simulink model "sm_car"  (R2025a)
settings: Solver=ode23t  StartTime=0.0  StopTime=400  MaxStep=0.4  RelTol=1e-3  AbsTol=1e-3  EnableMultiTasking=on
PreLoadFcn:
  | % Due to usability issue in Repeating Sequence block
  | warning('off','Simulink:Masking:Invalid');
  | 
  | % Eliminate unnecessary warnings in inactive variants
  | % Warnings generated only if you click through inactive variant
  | warning('off','MATLAB:nonExistentField');
  | warning('off','Simulink:Parameters:BlkParamUndefined');
PostLoadFcn:
  | set_param([bdroot '/Vehicle'],'popup_trailer','Off')
  | warning('off','sm:sli:setup:compile:LocalSolverNotSupported')
  | %sm_car_config_maneuver(bdroot,'WOT Braking');
  | sm_car_config_vehicle(bdroot,'false');
  | sm_car_config_logging(bdroot);
InitFcn:
  | sm_car_config_camera;
  | Vehicle = sm_car_vehcfg_checkConfig(Vehicle);
  | sm_car_check_tire_model(bdroot);
StartFcn:
  | tic;
StopFcn:
  | Elapsed_Sim_Time = toc;
  | % disp(['Elapsed Sim Time = ' num2str(Elapsed_Sim_Time)]);
undefined symbols (not defined in the file): Axle1D, AxleIn, Camera, Control, Driver, Free, Init, Maneuver, Pedal, RaceFix, RaceSpin, Scene, ShaftL1, ShaftL2, ShaftR1, ShaftR2, Soft, Stiff, Visual, X, xy_data_car_side, Y, Z
libraries: sm_lib x1546, nesl_utility x528, fl_lib x480, SimscapeFluids_lib x61, sdl_lib x49, simulink x29, ee_lib x7, simulink_extras x6, Linkage_Systems x4, Tire_1x2x x4, AntiRollBar_Systems x2, Linkage_Decoupled x2
(part 28 of 79)

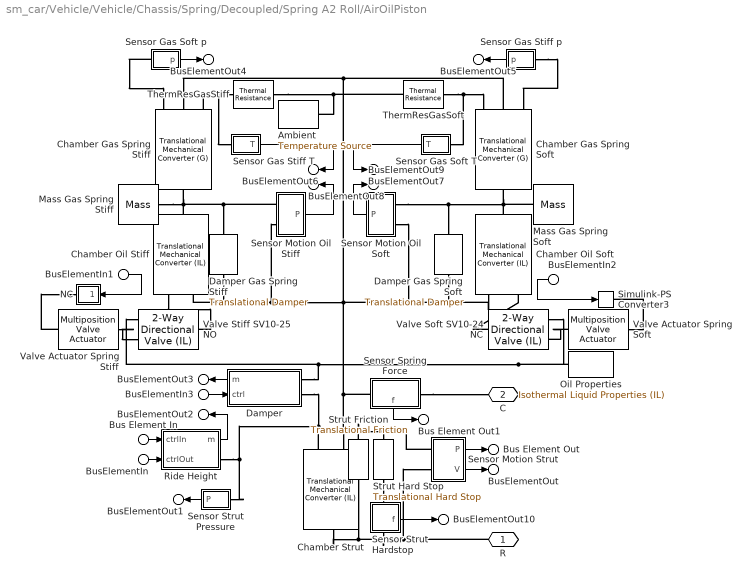
== system sm_car/Vehicle/Vehicle/Chassis/Spring/Decoupled/Spring A2 Roll/AirOilPiston ==
  BusElementIn1 : Inport  PortName=Ctrl  Element=GasSprStiff
  BusElementIn2 : Inport  PortName=Ctrl  Element=GasSprSoft
  BusElementIn3 : Inport  PortName=Ctrl  Element=Damper
  Bus Element In : Inport  PortName=Ctrl  Element=RideHeightIn
  BusElementIn : Inport  PortName=Ctrl  Element=RideHeightOut
  Ambient : fl_lib/Thermal/Thermal Sources/Temperature Source  temperature=t_ambient K
  Chamber Gas Spring Soft : fl_lib/Gas/Elements/Translational Mechanical Converter (G)  mech_orientation=foundation.enum.MechOrientationTranslational.Negative  displacement_spec=foundation.enum.DisplacementSpec.Calculate  length_init=gas_chamber_soft_x0 m  interface_area=gas_chamber_soft_area m^2  dead_volume=gas_chamber_soft_deadvol l  area_A=0.01 m^2  environment_spec=foundation.enum.pressure_spec.atmospheric  environment_pressure=0.101325 MPa  p_I_specify=on  p_I_priority=High  p_I=gas_chamber_soft_p0 MPa  p_I_nominal_specify=off  p_I_nominal_value=1  p_I_nominal_unit=MPa  T_I_specify=off  T_I_priority=High  T_I=293.15 K  T_I_nominal_specify=off  T_I_nominal_value=1  T_I_nominal_unit=K  rho_I_specify=off  rho_I_priority=None  rho_I=1.2 kg/m^3  rho_I_nominal_specify=off  rho_I_nominal_value=1  rho_I_nominal_unit=kg/m^3
      settings: InternalSimscapePortConfiguration="{\"Bottom\":[],\"Left\":[{\"id\":\"A\",\"label\":\"A\",\"type\":\"foundation.gas.gas\"},{\"id\":\"C\",\"label\":\"C\",\"type\":\"foundation.mechanical.translational.translational\"},{\"id\":\"H\",\"label\":\"H\",\"type\":\"foundation.thermal.thermal\"}],\"Right\":[{\"id\":\"R\",\"label\":\"R\",\"type\":\"foundation.mechanical.translational.translational\"}],\"Top\":[]}"
  Chamber Gas Spring Stiff : fl_lib/Gas/Elements/Translational Mechanical Converter (G)  mech_orientation=foundation.enum.MechOrientationTranslational.Negative  displacement_spec=foundation.enum.DisplacementSpec.Calculate  length_init=gas_chamber_stiff_x0 m  interface_area=gas_chamber_stiff_area m^2  dead_volume=gas_chamber_stiff_deadvol l  area_A=0.01 m^2  environment_spec=foundation.enum.pressure_spec.atmospheric  environment_pressure=0.101325 MPa  p_I_specify=on  p_I_priority=High  p_I=gas_chamber_stiff_p0 MPa  p_I_nominal_specify=off  p_I_nominal_value=1  p_I_nominal_unit=MPa  T_I_specify=off  T_I_priority=High  T_I=293.15 K  T_I_nominal_specify=off  T_I_nominal_value=1  T_I_nominal_unit=K  rho_I_specify=off  rho_I_priority=None  rho_I=1.2 kg/m^3  rho_I_nominal_specify=off  rho_I_nominal_value=1  rho_I_nominal_unit=kg/m^3
      settings: InternalSimscapePortConfiguration="{\"Bottom\":[],\"Left\":[{\"id\":\"A\",\"label\":\"A\",\"type\":\"foundation.gas.gas\"},{\"id\":\"C\",\"label\":\"C\",\"type\":\"foundation.mechanical.translational.translational\"},{\"id\":\"H\",\"label\":\"H\",\"type\":\"foundation.thermal.thermal\"}],\"Right\":[{\"id\":\"R\",\"label\":\"R\",\"type\":\"foundation.mechanical.translational.translational\"}],\"Top\":[]}"
  Chamber Oil Soft : fl_lib/Isothermal Liquid/Elements/Translational Mechanical Converter (IL)  mech_orientation=foundation.enum.MechOrientationTranslational.Positive  displacement_spec=foundation.enum.DisplacementSpec.Calculate  x0=oil_chamber_soft_x0 m  interface_area=oil_chamber_soft_area m^2  dead_volume=oil_chamber_soft_deadvol l  pressure_spec=foundation.enum.pressure_spec.atmospheric  environment_pressure=0.101325 MPa  dynamic_compressibility=simscape.enum.onoff.off  p0=Spring.Spring.OilSoft.pInit.Value MPa  p_nominal=0.101325 MPa
      settings: InternalSimscapePortConfiguration="{\"Bottom\":[],\"Left\":[{\"id\":\"A\",\"label\":\"A\",\"type\":\"foundation.isothermal_liquid.isothermal_liquid\"},{\"id\":\"C\",\"label\":\"C\",\"type\":\"foundation.mechanical.translational.translational\"}],\"Right\":[{\"id\":\"R\",\"label\":\"R\",\"type\":\"foundation.mechanical.translational.translational\"}],\"Top\":[]}"
  Chamber Oil Stiff : fl_lib/Isothermal Liquid/Elements/Translational Mechanical Converter (IL)  mech_orientation=foundation.enum.MechOrientationTranslational.Positive  displacement_spec=foundation.enum.DisplacementSpec.Calculate  x0=oil_chamber_stiff_x0 m  interface_area=oil_chamber_stiff_area m^2  dead_volume=oil_chamber_stiff_deadvol l  pressure_spec=foundation.enum.pressure_spec.atmospheric  environment_pressure=0.101325 MPa  dynamic_compressibility=simscape.enum.onoff.off  p0=Spring.Spring.OilStiff.pInit.Value MPa  p_nominal=0.101325 MPa
      settings: InternalSimscapePortConfiguration="{\"Bottom\":[],\"Left\":[{\"id\":\"A\",\"label\":\"A\",\"type\":\"foundation.isothermal_liquid.isothermal_liquid\"},{\"id\":\"C\",\"label\":\"C\",\"type\":\"foundation.mechanical.translational.translational\"}],\"Right\":[{\"id\":\"R\",\"label\":\"R\",\"type\":\"foundation.mechanical.translational.translational\"}],\"Top\":[]}"
  Chamber Strut : fl_lib/Isothermal Liquid/Elements/Translational Mechanical Converter (IL)  mech_orientation=foundation.enum.MechOrientationTranslational.Positive  displacement_spec=foundation.enum.DisplacementSpec.Calculate  x0=strut_x0 m  interface_area=strut_area m^2  dead_volume=strut_deadvol l  pressure_spec=foundation.enum.pressure_spec.atmospheric  environment_pressure=0.101325 MPa  dynamic_compressibility=simscape.enum.onoff.off  p0=P_initial MPa  p_nominal=0.101325 MPa
      settings: InternalSimscapePortConfiguration="{\"Bottom\":[],\"Left\":[{\"id\":\"A\",\"label\":\"A\",\"type\":\"foundation.isothermal_liquid.isothermal_liquid\"},{\"id\":\"C\",\"label\":\"C\",\"type\":\"foundation.mechanical.translational.translational\"}],\"Right\":[{\"id\":\"R\",\"label\":\"R\",\"type\":\"foundation.mechanical.translational.translational\"}],\"Top\":[]}"
  Damper : Subsystem  mask(Damper Module){p_diff_TLU_constant=p_diff_TLU_constant, vol_flow_TLU_constant=vol_flow_TLU_constant, dpr_restrarea_comp=dpr_restrarea_comp, dpr_restrarea_reb=dpr_restrarea_reb, dpr_cd_comp=dpr_cd_comp, dpr_cd_reb=dpr_cd_reb, dpr_prv_psetdiff_comp=dpr_prv_psetdiff_comp, dpr_prv_psetdiff_reb=dpr_prv_psetdiff_reb, dpr_prv_prange_comp=dpr_prv_prange_comp, dpr_prv_prange_reb=dpr_prv_prange_reb, dpr_prv_areamax_comp=dpr_prv_areamax_comp, dpr_prv_areamax_reb=dpr_prv_areamax_reb, dpr_prv_cd_comp=dpr_prv_cd_comp, dpr_prv_cd_reb=dpr_prv_cd_reb, dpr_cvdvalve_cmpos=dpr_cvdvalve_cmpos, dpr_cvdvalve_orifice_area=dpr_cvdvalve_orifice_area, dpr_cvdvalve_orifice_pdiff=dpr_cvdvalve_orifice_pdiff, dpr_cvdvalve_pcv_areamax=dpr_cvdvalve_pcv_areamax, dpr_cvdvalve_pcv_prange=dpr_cvdvalve_pcv_prange, dpr_cvdvalve_arealeak=dpr_cvdvalve_arealeak, dpr_cvdvalve_cd=dpr_cvdvalve_cd, dpr_cvdvalve_act_ts=dpr_cvdvalve_act_ts}
      mask prompts: p_diff_TLU_constant "Pressure Drop Vector (MPa)"; vol_flow_TLU_constant "Vol. Flow Rate (m^3/s)"; dpr_cvdvalve_cmpos "Orifice Pos. Vector (m)"; dpr_cvdvalve_orifice_area "Orifice Area (m^2)"; dpr_cvdvalve_orifice_pdiff "Orifice Set Press. Diff. (bar)"; dpr_cvdvalve_pcv_areamax "Pr. Comp. Valve Max Area (m^2)"; dpr_cvdvalve_pcv_prange "Pr. Comp. Valve Range (bar)"; dpr_cvdvalve_arealeak "Leakage Area (m^2)"; dpr_cvdvalve_cd "Discharge Coeff (Cd)"; dpr_cvdvalve_act_ts "Actuator Time Constant (s)"
      mask help: Models damper module with multiple flow paths. Low-speed damping characteristic modeled with an orifice. Unique rebound and compression characteristics modeled with pressure-relief valves. Dynamic control of damping modeled with a pressure compensated flow control valve.
      settings: PortSchema="{\"entries\":[{\"content\":{\"sides\":[{\"content\":{},\"type\":\"ConnectorPlacement.EquallySpacedRectSide\",\"uuid\":\"a5f791c8-acac-4d53-8c58-1049a1347491\"},{\"content\":{\"side\":\"RIGHT\"},\"type\":\"ConnectorPlacement.EquallySpacedRectSide\",\"uuid\":\"abd68a62-c541-4b1e-beea-443f2561f93e\"},{\"content\":{\"connectorIds\":[\"LConn1\",\"LConn2\"],\"side\":\"TOP\"},\"type\":\"ConnectorPlacement.EquallySpacedRectSide\",\"uuid\":\"a9a9664c-7859-4d06-89f2-97c7cf0d89ed\"},{\"content\":{\"connectorIds\":[\"In1\",\"Out1\"],\"side\":\"BOTTOM\"},\"type\":\"ConnectorPlacement.EquallySpacedRectSide\",\"uuid\":\"7b16d6fa-efa2-4cfe-ba47-347a90763739\"}]},\"type\":\"ConnectorPlacement.EquallySpacedConnector\",\"uuid\":\"a3eac46d-3875-4d11-90c1-dfb44d5e1ceb\"}],\"packageUris\":[\"http://schema.mathworks.com/mf0/Connector/R2020b\"],\"version\":\"1.0\"}"
      mask TypeOptions p_diff_TLU_constant: Orifice Low Speed/p_diff_TLU_constant
      mask TypeOptions vol_flow_TLU_constant: Orifice Low Speed/vol_flow_TLU_constant
      mask TypeOptions dpr_restrarea_comp: Restr Comp/restriction_area
      mask TypeOptions dpr_restrarea_reb: Restr Reb/restriction_area
      mask TypeOptions dpr_cd_comp: Restr Comp/Cd
      mask TypeOptions dpr_cd_reb: Restr Reb/Cd
      mask TypeOptions dpr_prv_psetdiff_comp: PRV Comp/p_set_differential
      mask TypeOptions dpr_prv_psetdiff_reb: PRV Reb/p_set_differential
      mask TypeOptions dpr_prv_prange_comp: PRV Reb/p_range
      mask TypeOptions dpr_prv_prange_reb: PRV Comp/p_range
      mask TypeOptions dpr_prv_areamax_comp: PRV Comp/area_max
      mask TypeOptions dpr_prv_areamax_reb: PRV Reb/area_max
      mask TypeOptions dpr_prv_cd_comp: PRV Comp/Cd
      mask TypeOptions dpr_prv_cd_reb: PRV Reb/Cd
      mask TypeOptions dpr_cvdvalve_cmpos: CVD Valve/S_TLU
      mask TypeOptions dpr_cvdvalve_orifice_area: CVD Valve/orifice_area_TLU
      mask TypeOptions dpr_cvdvalve_orifice_pdiff: CVD Valve/p_diff_orifice
      mask TypeOptions dpr_cvdvalve_pcv_areamax: CVD Valve/area_max_compensator
      mask TypeOptions dpr_cvdvalve_pcv_prange: CVD Valve/p_range
      mask TypeOptions dpr_cvdvalve_arealeak: CVD Valve/area_leak
      mask TypeOptions dpr_cvdvalve_cd: CVD Valve/Cd
      mask TypeOptions dpr_cvdvalve_act_ts: CVD Actuator/time_constant
      mask DialogControl tab_damper Prompt: Damper
      mask DialogControl cont_orifice_ls Prompt: Low Speed Orifice
      mask DialogControl cont_blowoff_restriction Prompt: Blowoff Restriction
      mask DialogControl text_blowoff_comp Prompt: Compression
      mask DialogControl text_blowoff_reb Prompt: Rebound
      mask DialogControl text_restr_area Prompt: Restr. Area (m^2)
      mask DialogControl text_cd Prompt: Cd
      mask DialogControl cont_blowoff_prv Prompt: Blowoff PRV
      mask DialogControl text_blowoff_prv_comp Prompt: Compression
      mask DialogControl text_blowoff_prv_reb Prompt: Rebound
      mask DialogControl text_psetdiff Prompt: Press. Diff. (MPa)
      mask DialogControl text_prange Prompt: Press. Range (MPa)
      mask DialogControl text_areamax Prompt: Max Area (m^2)
      mask DialogControl text_blowoff_cd Prompt: Cd
      mask DialogControl cont_dpr_cvd_valve Prompt: CVD Valve
  Damper Gas Spring Soft : sdl_lib/Couplings & Drives/Springs & Dampers/Translational Damper  D=gspr_damping_soft N*s/m  thermal_port=simscape.enum.thermaleffects.omit  thermal_mass=50 kJ/K  temperature_specify=off  temperature_priority=High  temperature=300 K  temperature_nominal_specify=off  temperature_nominal_value=1  temperature_nominal_unit=K
  "Damper Gas Spring Stiff " : sdl_lib/Couplings & Drives/Springs & Dampers/Translational Damper  D=gspr_damping_stiff N*s/m  thermal_port=simscape.enum.thermaleffects.omit  thermal_mass=50 kJ/K  temperature_specify=off  temperature_priority=High  temperature=300 K  temperature_nominal_specify=off  temperature_nominal_value=1  temperature_nominal_unit=K
  Mass Gas Spring Soft : fl_lib/Mechanical/Translational Elements/Mass  mass=gspr_mass_soft kg  num_ports=foundation.enum.numPorts2.one  v_specify=off  v_priority=High  v=0 m/s  v_nominal_specify=off  v_nominal_value=1  v_nominal_unit=m/s  f_specify=off  f_priority=None  f=0 N  f_nominal_specify=off  f_nominal_value=1  f_nominal_unit=N
  Mass Gas Spring Stiff : fl_lib/Mechanical/Translational Elements/Mass  mass=gspr_mass_stiff kg  num_ports=foundation.enum.numPorts2.one  v_specify=off  v_priority=High  v=0 m/s  v_nominal_specify=off  v_nominal_value=1  v_nominal_unit=m/s  f_specify=off  f_priority=None  f=0 N  f_nominal_specify=off  f_nominal_value=1  f_nominal_unit=N
  NC : Subsystem
  Oil Properties : fl_lib/Isothermal Liquid/Utilities/Isothermal Liquid Properties (IL)  rho_L_atm=oilprop_rho kg/m^3  bulk_modulus_model=foundation.enum.bulk_modulus_model.const  beta_gain=6  beta_L_atm=oilprop_B Pa  nu_atm=oilprop_nu cSt  p_atm=0.101325 MPa  p_min=0.001 Pa  properties_range_check=simscape.enum.assert.action.error  air_fraction=0.005  polytropic_index=1.0  rho_g_atm=1.225 kg/m^3  air_dissolution_model=simscape.enum.onoff.off  p_crit=3 MPa
  Ride Height : Subsystem  mask(Ride Height Adjustment System){rh_srcpressure=rh_srcpressure, rh_fcv_cmpos_inlet=rh_fcv_cmpos_inlet, rh_fcv_cmpos_outlet=rh_fcv_cmpos_outlet, rh_fcv_orificearea_inlet=rh_fcv_orificearea_inlet, rh_fcv_orificearea_outlet=rh_fcv_orificearea_outlet, rh_fcv_orificepdiff_inlet=rh_fcv_orificepdiff_inlet, rh_fcv_orificepdiff_outlet=rh_fcv_orificepdiff_outlet, rh_fcv_pcprange_inlet=rh_fcv_pcprange_inlet, rh_fcv_pcprange_outlet=rh_fcv_pcprange_outlet, rh_fcv_pcamax_inlet=rh_fcv_pcamax_inlet, rh_fcv_pcamax_outlet=rh_fcv_pcamax_outlet, rh_fcv_arealeak_inlet=rh_fcv_arealeak_inlet, rh_fcv_arealeak_outlet=rh_fcv_arealeak_outlet, rh_fcv_cd_inlet=rh_fcv_cd_inlet, rh_fcv_cd_outlet=rh_fcv_cd_outlet, rh_fcv_smooth_inlet=rh_fcv_smooth_inlet, rh_fcv_smooth_outlet=rh_fcv_smooth_outlet, rh_fcv_tfilt_inlet=rh_fcv_tfilt_inlet, rh_fcv_tfilt_outlet=rh_fcv_tfilt_outlet}
      mask prompts: rh_srcpressure "Source Pressure (MPa)"
      mask help: Models ride height adjustment system. Valves control oil flow to the lower oil chamber.
      mask TypeOptions rh_srcpressure: Pressure Source (IL)/pressure_differential
      mask TypeOptions rh_fcv_cmpos_inlet: FCV Inlet/S_TLU
      mask TypeOptions rh_fcv_cmpos_outlet: FCV Outlet/S_TLU
      mask TypeOptions rh_fcv_orificearea_inlet: FCV Inlet/orifice_area_TLU
      mask TypeOptions rh_fcv_orificearea_outlet: FCV Outlet/orifice_area_TLU
      mask TypeOptions rh_fcv_orificepdiff_inlet: FCV Inlet/p_diff_orifice
      mask TypeOptions rh_fcv_orificepdiff_outlet: FCV Outlet/p_diff_orifice
      mask TypeOptions rh_fcv_pcprange_inlet: FCV Inlet/p_range
      mask TypeOptions rh_fcv_pcprange_outlet: FCV Outlet/p_range
      mask TypeOptions rh_fcv_pcamax_inlet: FCV Inlet/area_max_compensator
      mask TypeOptions rh_fcv_pcamax_outlet: FCV Outlet/area_max_compensator
      mask TypeOptions rh_fcv_arealeak_inlet: FCV Inlet/area_leak
      mask TypeOptions rh_fcv_arealeak_outlet: FCV Outlet/area_leak
      mask TypeOptions rh_fcv_cd_inlet: FCV Inlet/Cd
      mask TypeOptions rh_fcv_cd_outlet: FCV Outlet/Cd
      mask TypeOptions rh_fcv_smooth_inlet: FCV Inlet/smoothing_factor
      mask TypeOptions rh_fcv_smooth_outlet: FCV Outlet/smoothing_factor
      mask TypeOptions rh_fcv_tfilt_inlet: FCV Actuator Inlet/time_constant
      mask TypeOptions rh_fcv_tfilt_outlet: FCV Actuator Outlet/time_constant
      mask DialogControl tab_ride_height Prompt: Ride Height
      mask DialogControl text_rideheight_inlet Prompt: Inlet
      mask DialogControl text_rideheight_outlet Prompt: Outlet
      mask DialogControl text_rh_fcv_cmpos Prompt: Orifice Pos. Vec. (m)
      mask DialogControl text_rh_fcv_orificearea Prompt: Orifice Area Vec (m^2)
      mask DialogControl text_rh_fcv_orificepdiff Prompt: Orifice Pr. Diff (bar)
      mask DialogControl text_rh_fcv_pcprange Prompt: Pr. Comp. Range (bar)
      mask DialogControl text_rh_fcv_pcamax Prompt: Pr. Comp. A Max (m^2)
      mask DialogControl text_rh_fcv_arealeak Prompt: Leakage Area (m^2)
      mask DialogControl text_rh_fcv_cd Prompt: Cd
      mask DialogControl text_rh_fcv_smooth Prompt: Smoothing
      mask DialogControl text_rh_fcv_tfilt Prompt: Time Constant (s)
  Sensor Motion Oil Soft : Subsystem
  Sensor Motion Oil Stiff : Subsystem
  Sensor Strut Hardstop : Subsystem
      settings: PortSchema="{\"entries\":[{\"content\":{\"sides\":[{\"content\":{\"connectorIds\":[\"LConn1\"]},\"type\":\"ConnectorPlacement.EquallySpacedRectSide\",\"uuid\":\"bda0782d-d0fc-4b4b-b54e-422fd5cad923\"},{\"content\":{\"connectorIds\":[\"RConn1\"],\"side\":\"RIGHT\"},\"type\":\"ConnectorPlacement.EquallySpacedRectSide\",\"uuid\":\"118fd084-4d20-4807-bd09-529e84dee962\"},{\"content\":{\"side\":\"TOP\"},\"type\":\"ConnectorPlacement.EquallySpacedRectSide\",\"uuid\":\"7375e241-c6a2-4517-b519-f2189b6a2bdc\"},{\"content\":{\"connectorIds\":[\"Out1\"],\"side\":\"BOTTOM\"},\"type\":\"ConnectorPlacement.EquallySpacedRectSide\",\"uuid\":\"8ffc5929-ef00-4e3f-aafa-18eff432822b\"}]},\"type\":\"ConnectorPlacement.EquallySpacedConnector\",\"uuid\":\"d009ba7a-74b3-470e-969a-6de4a504fd4b\"}],\"packageUris\":[\"http://schema.mathworks.com/mf0/Connector/R2020b\"],\"version\":\"1.0\"}"
  Sensor Gas Soft T : Subsystem
  Sensor Gas Soft p : Subsystem
  "Sensor Gas Stiff T " : Subsystem
  Sensor Gas Stiff p : Subsystem
  Sensor Motion Strut : Subsystem
  Sensor Spring Force : Subsystem
      settings: PortSchema="{\"entries\":[{\"content\":{\"sides\":[{\"content\":{\"connectorIds\":[\"LConn1\"]},\"type\":\"ConnectorPlacement.EquallySpacedRectSide\",\"uuid\":\"bda0782d-d0fc-4b4b-b54e-422fd5cad923\"},{\"content\":{\"connectorIds\":[\"RConn1\"],\"side\":\"RIGHT\"},\"type\":\"ConnectorPlacement.EquallySpacedRectSide\",\"uuid\":\"118fd084-4d20-4807-bd09-529e84dee962\"},{\"content\":{\"side\":\"TOP\"},\"type\":\"ConnectorPlacement.EquallySpacedRectSide\",\"uuid\":\"7375e241-c6a2-4517-b519-f2189b6a2bdc\"},{\"content\":{\"connectorIds\":[\"Out1\"],\"side\":\"BOTTOM\"},\"type\":\"ConnectorPlacement.EquallySpacedRectSide\",\"uuid\":\"73d23305-f348-4909-b09c-dbea63020875\"}]},\"type\":\"ConnectorPlacement.EquallySpacedConnector\",\"uuid\":\"d009ba7a-74b3-470e-969a-6de4a504fd4b\"}],\"packageUris\":[\"http://schema.mathworks.com/mf0/Connector/R2020b\"],\"version\":\"1.0\"}"
  Sensor Strut Pressure : Subsystem
  Simulink-PS Converter3 : nesl_utility/Simulink-PS Converter  PhysicalDomain=network_engine_domain  SubClassName=ps_input  LeftPortType=input  RightPortType=output  PseudoPeriodic=off  Frequencies=[]  NoiseDistribution=none  NoiseParameters=[]  Unit=1  AffineConversion=off  FilteringAndDerivatives=provide  SimscapeFilterOrder=1  InputFilterTimeConstant=0.001  UdotUserProvided=0
  Strut Friction : fl_lib/Mechanical/Translational Elements/Translational Friction  brkwy_frc=strut_frc_brkfrc N  brkwy_vel=strut_frc_brkvel m/s  Col_frc=strut_frc_colfrc N  visc_coef=strut_frc_visccoeff N*s/m  v_specify=off  v_priority=None  v=0 m/s  v_nominal_specify=off  v_nominal_value=1  v_nominal_unit=m/s  f_specify=off  f_priority=None  f=0 N  f_nominal_specify=off  f_nominal_value=1  f_nominal_unit=N
      settings: InternalSimscapePortConfiguration="{\"Bottom\":[],\"Left\":[{\"id\":\"R\",\"label\":\"R\",\"type\":\"foundation.mechanical.translational.translational\"}],\"Right\":[{\"id\":\"C\",\"label\":\"C\",\"type\":\"foundation.mechanical.translational.translational\"}],\"Top\":[]}"
  Strut Hard Stop : fl_lib/Mechanical/Translational Elements/Translational Hard Stop  upper_bnd=bs_lim_upper m  lower_bnd=bs_lim_lower m  model=simscape.enum.hardstop.smooth  stiff_up=bs_k_upper N/m  stiff_low=bs_k_lower N/m  D_up=bs_b_upper N*s/m  D_low=bs_b_lower N*s/m  transition=bs_region mm  coeff_rest=0.7  v_tol=0.001 m/s  f_tol=0.001 N  v_specify=off  v_priority=None  v=0 m/s  v_nominal_specify=off  v_nominal_value=1  v_nominal_unit=m/s  f_specify=off  f_priority=None  f=0 N  f_nominal_specify=off  f_nominal_value=1  f_nominal_unit=N  x_specify=off  x_priority=High  x=0 m  x_nominal_specify=off  x_nominal_value=1  x_nominal_unit=m  M_specify=off  M_priority=None  M=0
  ThermResGasSoft : fl_lib/Thermal/Thermal Elements/Thermal Resistance  resistance=gspr_cwall_soft K/W  T_specify=off  T_priority=None  T=0 K  T_nominal_specify=off  T_nominal_value=1  T_nominal_unit=K  Q_specify=off  Q_priority=None  Q=0 W  Q_nominal_specify=off  Q_nominal_value=1  Q_nominal_unit=W
  ThermResGasStiff : fl_lib/Thermal/Thermal Elements/Thermal Resistance  resistance=gspr_cwall_stiff K/W  T_specify=off  T_priority=None  T=0 K  T_nominal_specify=off  T_nominal_value=1  T_nominal_unit=K  Q_specify=off  Q_priority=None  Q=0 W  Q_nominal_specify=off  Q_nominal_value=1  Q_nominal_unit=W
  Valve Actuator Spring Soft : SimscapeFluids_lib/Valve Actuators/Multiposition Valve Actuator  positions=fluids.valve_actuators.enum.actuator_num_positions.two  stroke=gsprva_stroke_soft m  t_on=gsprva_ton_soft s  t_off=gsprva_toff_soft s  act_signal=1  init_position_2=fluids.valve_actuators.enum.actuator_two_pos_ic.extended  init_position_3=fluids.valve_actuators.enum.actuator_three_pos_ic.neutral  act_orientation=simscape.enum.posneg.positive  local_time_specify=off  local_time_priority=None  local_time=0 s  local_time_nominal_specify=off  local_time_nominal_value=1  local_time_nominal_unit=s
      settings: InternalSimscapePortConfiguration="{\"Bottom\":[],\"Left\":[{\"id\":\"A\",\"label\":\"A\",\"type\":\"input\"}],\"Right\":[{\"id\":\"S\",\"label\":\"S\",\"type\":\"output\"}],\"Top\":[]}"
  Valve Actuator Spring Stiff : SimscapeFluids_lib/Valve Actuators/Multiposition Valve Actuator  positions=fluids.valve_actuators.enum.actuator_num_positions.two  stroke=gsprva_stroke_stiff m  t_on=gsprva_ton_stiff s  t_off=gsprva_toff_stiff s  act_signal=1  init_position_2=fluids.valve_actuators.enum.actuator_two_pos_ic.extended  init_position_3=fluids.valve_actuators.enum.actuator_three_pos_ic.neutral  act_orientation=simscape.enum.posneg.positive  local_time_specify=off  local_time_priority=None  local_time=0 s  local_time_nominal_specify=off  local_time_nominal_value=1  local_time_nominal_unit=s
      settings: InternalSimscapePortConfiguration="{\"Bottom\":[],\"Left\":[{\"id\":\"A\",\"label\":\"A\",\"type\":\"input\"}],\"Right\":[{\"id\":\"S\",\"label\":\"S\",\"type\":\"output\"}],\"Top\":[]}"
  Valve Soft SV10-24 NC : SimscapeFluids_lib/Isothermal Liquid/Valves & Orifices/Directional Control Valves/2-Way Directional Valve (IL)  valve_spec=fluids.isothermal_liquid.valves_orifices.directional_control_valves.enum.directional_valve_spec.linear  S_max=gsprv_smax_soft m  del_S_max=gsprv_delsmax_soft m  area_max=gsprv_areamax_soft m^2  area_leak=gsprv_arealeak_soft m^2  del_S_TLU=[0, .002, .004, .007, .017] m  orifice_area_TLU=[1e-09, 2.0352e-07, 4.0736e-05, .00011438, .00034356] m^2  del_S_vol_flow_TLU=[0, .002, .004, .007, .017] m  p_diff_TLU=[.3, .5, .7] MPa  vol_flow_TLU=1e-3 * [1.7e-05, 2e-05, 2.6e-05; .0035, .0045, .0053; .7, .9, 1.06; 1.96, 2.5, 3; 6, 7.7, 9.13] m^3/s  Cd=gsprv_cd_soft  Re_c=150  smoothing_factor=gsprv_smooth_soft  pressure_recovery=simscape.enum.onoff.off  area=inf m^2
      settings: InternalSimscapePortConfiguration="{\"Bottom\":[{\"id\":\"B\",\"label\":\"B\",\"type\":\"foundation.isothermal_liquid.isothermal_liquid\"}],\"Left\":[{\"id\":\"S\",\"label\":\"S\",\"type\":\"input\"}],\"Right\":[],\"Top\":[{\"id\":\"A\",\"label\":\"A\",\"type\":\"foundation.isothermal_liquid.isothermal_liquid\"}]}"
  Valve Stiff SV10-25 NO : SimscapeFluids_lib/Isothermal Liquid/Valves & Orifices/Directional Control Valves/2-Way Directional Valve (IL)  valve_spec=fluids.isothermal_liquid.valves_orifices.directional_control_valves.enum.directional_valve_spec.linear  S_max=gsprv_smax_stiff m  del_S_max=gsprv_delsmax_stiff m  area_max=gsprv_areamax_stiff m^2  area_leak=gsprv_arealeak_stiff m^2  del_S_TLU=[0, .002, .004, .007, .017] m  orifice_area_TLU=[1e-09, 2.0352e-07, 4.0736e-05, .00011438, .00034356] m^2  del_S_vol_flow_TLU=[0, .002, .004, .007, .017] m  p_diff_TLU=[.3, .5, .7] MPa  vol_flow_TLU=1e-3 * [1.7e-05, 2e-05, 2.6e-05; .0035, .0045, .0053; .7, .9, 1.06; 1.96, 2.5, 3; 6, 7.7, 9.13] m^3/s  Cd=gsprv_cd_stiff  Re_c=150  smoothing_factor=gsprv_smooth_stiff  pressure_recovery=simscape.enum.onoff.off  area=inf m^2
      settings: InternalSimscapePortConfiguration="{\"Bottom\":[{\"id\":\"B\",\"label\":\"B\",\"type\":\"foundation.isothermal_liquid.isothermal_liquid\"}],\"Left\":[{\"id\":\"S\",\"label\":\"S\",\"type\":\"input\"}],\"Right\":[],\"Top\":[{\"id\":\"A\",\"label\":\"A\",\"type\":\"foundation.isothermal_liquid.isothermal_liquid\"}]}"
  R : PMIOPort  Side=Left
  C : PMIOPort  Port=2  Side=Right
  BusElementOut3 : Outport  PortName=meas  Element=Damper
  BusElementOut6 : Outport  PortName=meas  Element=GasSprStiff.T
  BusElementOut8 : Outport  PortName=meas  Element=GasSprStiff.x
  BusElementOut4 : Outport  PortName=meas  Element=GasSprStiff.P
  BusElementOut5 : Outport  PortName=meas  Element=GasSprSoft.P
  BusElementOut7 : Outport  PortName=meas  Element=GasSprSoft.T
  BusElementOut9 : Outport  PortName=meas  Element=GasSprSoft.x
  BusElementOut1 : Outport  PortName=meas  Element=Strut.P
  BusElementOut2 : Outport  PortName=meas  Element=RideHeight
  Bus Element Out : Outport  PortName=meas  Element=xSpring
  BusElementOut : Outport  PortName=meas  Element=vSpring
  Bus Element Out1 : Outport  PortName=meas  Element=FSpring
  BusElementOut10 : Outport  PortName=meas  Element=FBumpstop
  wires:
  BusElementIn3/1 -> Damper/1(ctrl)
  Sensor Motion Oil Stiff/1(P) -> BusElementOut8/1
  Sensor Gas Soft p/1(p) -> BusElementOut4/1
  Sensor Gas Stiff p/1(p) -> BusElementOut5/1
  BusElementIn1/1 -> NC/1(c)
  BusElementIn2/1 -> Simulink-PS Converter3/1
  Damper/1(m) -> BusElementOut3/1
  "Sensor Gas Stiff T "/1(T) -> BusElementOut6/1
  Sensor Gas Soft T/1(T) -> BusElementOut7/1
  Sensor Motion Oil Soft/1(P) -> BusElementOut9/1
  Sensor Motion Strut/1(P) -> Bus Element Out/1
  Sensor Motion Strut/2(V) -> BusElementOut/1
  Bus Element In/1 -> Ride Height/1(ctrlIn)
  BusElementIn/1 -> Ride Height/2(ctrlOut)
  Sensor Strut Pressure/1(P) -> BusElementOut1/1
  Ride Height/1(m) -> BusElementOut2/1
  Sensor Spring Force/1(f) -> Bus Element Out1/1
  Sensor Strut Hardstop/1(f) -> BusElementOut10/1
  connections:
  Damper/LConn2 -- Valve Stiff SV10-25 NO/LConn2 -- Valve Soft SV10-24 NC/LConn2 -- Oil Properties/RConn1
  ThermResGasStiff/RConn1 -- ThermResGasSoft/RConn1 -- Ambient/LConn1
  Chamber Oil Stiff/RConn1 -- Sensor Motion Oil Stiff/LConn1 -- "Damper Gas Spring Stiff "/LConn1 -- Mass Gas Spring Stiff/LConn1 -- Chamber Gas Spring Stiff/RConn1
  Sensor Gas Soft p/LConn1 -- Chamber Gas Spring Stiff/LConn1
  Chamber Gas Spring Stiff/LConn3 -- "Sensor Gas Stiff T "/LConn1 -- ThermResGasStiff/LConn1
  Chamber Oil Stiff/LConn1 -- Valve Stiff SV10-25 NO/RConn1
  Valve Actuator Spring Stiff/RConn1 -- Valve Stiff SV10-25 NO/LConn1
  Valve Actuator Spring Stiff/LConn1 -- NC/RConn1
  Chamber Oil Soft/RConn1 -- Mass Gas Spring Soft/LConn1 -- Sensor Motion Oil Soft/LConn1 -- Damper Gas Spring Soft/LConn1 -- Chamber Gas Spring Soft/RConn1
  Sensor Gas Stiff p/LConn1 -- Chamber Gas Spring Soft/LConn1
  ThermResGasSoft/LConn1 -- Sensor Gas Soft T/LConn1 -- Chamber Gas Spring Soft/LConn3
  Valve Soft SV10-24 NC/RConn1 -- Chamber Oil Soft/LConn1
  Valve Actuator Spring Soft/RConn1 -- Valve Soft SV10-24 NC/LConn1
  Valve Actuator Spring Soft/LConn1 -- Simulink-PS Converter3/RConn1
  Chamber Strut/RConn1 -- Sensor Strut Hardstop/RConn1 -- R/RConn1 -- Sensor Motion Strut/LConn2 -- Strut Friction/LConn1
  Damper/LConn1 -- Sensor Strut Pressure/LConn1 -- Ride Height/RConn1 -- Chamber Strut/LConn1
  Strut Hard Stop/LConn1 -- Sensor Strut Hardstop/LConn1
  Chamber Oil Soft/LConn2 -- Damper Gas Spring Soft/RConn1 -- Sensor Motion Oil Soft/LConn2 -- Strut Friction/RConn1 -- Sensor Motion Strut/LConn1 -- Strut Hard Stop/RConn1 -- Chamber Strut/LConn2 -- Sensor Spring Force/RConn1 -- Chamber Gas Spring Stiff/LConn2 -- Chamber Gas Spring Soft/LConn2 -- "Damper Gas Spring Stiff "/RConn1 -- Chamber Oil Stiff/LConn2 -- Sensor Motion Oil Stiff/LConn2
  Sensor Spring Force/LConn1 -- C/RConn1

== system sm_car/Vehicle/Vehicle/Chassis/Spring/Decoupled/Spring A2 Roll/Linear ==
  note: Sensing
  Ctrl : Inport
  Displacement Spring : fl_lib/Mechanical/Mechanical Sensors/Ideal Translational Motion Sensor  reference=foundation.enum.MeasurementReference.difference  acceleration_port=false  velocity_port=true  position_port=true  offset=spr_len0 m
  Force Spring : fl_lib/Mechanical/Mechanical Sensors/Ideal Force Sensor
  PS Term Motion v : fl_lib/Physical Signals/Sinks/PS Terminator
  PS-Simulink Converter : nesl_utility/PS-Simulink Converter  PhysicalDomain=network_engine_domain  SubClassName=ps_output  LeftPortType=input  RightPortType=output  PseudoPeriodic=off  Frequencies=[]  VectorFormat=1-D array  Unit=m  AffineConversion=off
  PS-Simulink Converter1 : nesl_utility/PS-Simulink Converter  PhysicalDomain=network_engine_domain  SubClassName=ps_output  LeftPortType=input  RightPortType=output  PseudoPeriodic=off  Frequencies=[]  VectorFormat=1-D array  Unit=N  AffineConversion=off
  Spring : fl_lib/Mechanical/Translational Elements/Translational Spring  spr_rate=spr_k N/m  v_specify=off  v_priority=None  v=0 m/s  v_nominal_specify=off  v_nominal_value=1  v_nominal_unit=m/s  f_specify=on  f_priority=High  f=-spr_frc0 N  f_nominal_specify=off  f_nominal_value=1  f_nominal_unit=N  x_specify=on  x_priority=None  x=-spr_def0 m  x_nominal_specify=off  x_nominal_value=1  x_nominal_unit=m
  Terminator : Terminator
  R : PMIOPort  Side=Left
  C : PMIOPort  Port=2  Side=Right
  Out Bus Element : Outport  VectorParamsAs1DForOutWhenUnconnected=off  PortName=meas  Element=xSpring
  Out Bus Element1 : Outport  VectorParamsAs1DForOutWhenUnconnected=off  PortName=meas  Element=FSpring
  wires:
  PS-Simulink Converter1/1 -> Out Bus Element1/1
  Ctrl/1 -> Terminator/1
  PS-Simulink Converter/1 -> Out Bus Element/1
  connections:
  Spring/LConn1 -- R/RConn1 -- Displacement Spring/LConn1
  Spring/RConn1 -- Force Spring/RConn1 -- Displacement Spring/RConn1
  Force Spring/LConn1 -- C/RConn1
  PS-Simulink Converter1/LConn1 -- Force Spring/RConn2
  Displacement Spring/RConn2 -- PS Term Motion v/LConn1
  Displacement Spring/RConn3 -- PS-Simulink Converter/LConn1

== system sm_car/Vehicle/Vehicle/Chassis/Spring/Decoupled/Spring A2 Roll/No Spring ==
  note: Sensor inserted simply to ensure
      | all blocks are connected to a network
  Ctrl : Inport
  Constant : Constant  Value=0
  Constant1 : Constant  Value=0
  Ideal Translational Motion Sensor : fl_lib/Mechanical/Mechanical Sensors/Ideal Translational Motion Sensor  reference=foundation.enum.MeasurementReference.difference  acceleration_port=false  velocity_port=true  position_port=true  offset=0 m
  PS-Simulink Converter : nesl_utility/PS-Simulink Converter  PhysicalDomain=network_engine_domain  SubClassName=ps_output  LeftPortType=input  RightPortType=output  PseudoPeriodic=off  Frequencies=[]  VectorFormat=1-D array  Unit=1  AffineConversion=off
  PS-Simulink Converter1 : nesl_utility/PS-Simulink Converter  PhysicalDomain=network_engine_domain  SubClassName=ps_output  LeftPortType=input  RightPortType=output  PseudoPeriodic=off  Frequencies=[]  VectorFormat=1-D array  Unit=1  AffineConversion=off
  Terminator : Terminator
  Terminator1 : Terminator
  Terminator2 : Terminator
  R : PMIOPort  Side=Left
  C : PMIOPort  Port=2  Side=Right
  Out Bus Element : Outport  VectorParamsAs1DForOutWhenUnconnected=off  PortName=meas  Element=xSpring
  Out Bus Element1 : Outport  VectorParamsAs1DForOutWhenUnconnected=off  PortName=meas  Element=FSpring
  wires:
  PS-Simulink Converter/1 -> Terminator1/1
  PS-Simulink Converter1/1 -> Terminator2/1
  Constant1/1 -> Out Bus Element/1
  Ctrl/1 -> Terminator/1
  Constant/1 -> Out Bus Element1/1
  connections:
  Ideal Translational Motion Sensor/RConn2 -- PS-Simulink Converter/LConn1
  PS-Simulink Converter1/LConn1 -- Ideal Translational Motion Sensor/RConn3
  C/RConn1 -- Ideal Translational Motion Sensor/RConn1
  R/RConn1 -- Ideal Translational Motion Sensor/LConn1

== system sm_car/Vehicle/Vehicle/Chassis/Spring/Decoupled/Spring A2 Roll/Nonlinear ==
  note: Sensing
  Ctrl : Inport
  Displacement Spring : fl_lib/Mechanical/Mechanical Sensors/Ideal Translational Motion Sensor  reference=foundation.enum.MeasurementReference.difference  acceleration_port=false  velocity_port=true  position_port=true  offset=spr_len0 m
  Force Spring : fl_lib/Mechanical/Mechanical Sensors/Ideal Force Sensor
  PS Term Motion v : fl_lib/Physical Signals/Sinks/PS Terminator
  PS-Simulink Converter : nesl_utility/PS-Simulink Converter  PhysicalDomain=network_engine_domain  SubClassName=ps_output  LeftPortType=input  RightPortType=output  PseudoPeriodic=off  Frequencies=[]  VectorFormat=1-D array  Unit=m  AffineConversion=off
  PS-Simulink Converter1 : nesl_utility/PS-Simulink Converter  PhysicalDomain=network_engine_domain  SubClassName=ps_output  LeftPortType=input  RightPortType=output  PseudoPeriodic=off  Frequencies=[]  VectorFormat=1-D array  Unit=N  AffineConversion=off
  Spring : sdl_lib/Couplings & Drives/Springs & Dampers/Nonlinear Translational Spring  parameterization=2  symmetry=1  coefficient_vector=[100, 0, 10, 0, 1] N/m  tension_coefficient_vector=[100, 0, 10, 0, 1] N/m  compression_coefficient_vector=[1000, -10, 100, 0, 0] N/m  deformation_vector=deformation_vector m  force_vector=force_vector N  interp_method=simscape.enum.interpolation.linear  extrap_method=simscape.enum.extrapolation.linear  x_specify=on  x_priority=High  x=spr_x0 m  x_nominal_specify=off  x_nominal_value=1  x_nominal_unit=m
      settings: InternalSimscapePortConfiguration="{\"Bottom\":[],\"Left\":[{\"id\":\"R\",\"label\":\"R\",\"type\":\"foundation.mechanical.translational.translational\"}],\"Right\":[{\"id\":\"C\",\"label\":\"C\",\"type\":\"foundation.mechanical.translational.translational\"}],\"Top\":[]}"
  Terminator : Terminator
  R : PMIOPort  Side=Left
  C : PMIOPort  Port=2  Side=Right
  Out Bus Element : Outport  VectorParamsAs1DForOutWhenUnconnected=off  PortName=meas  Element=xSpring
  Out Bus Element1 : Outport  VectorParamsAs1DForOutWhenUnconnected=off  PortName=meas  Element=FSpring
  wires:
  PS-Simulink Converter/1 -> Out Bus Element/1
  Ctrl/1 -> Terminator/1
  PS-Simulink Converter1/1 -> Out Bus Element1/1
  connections:
  Displacement Spring/RConn3 -- PS-Simulink Converter/LConn1
  Displacement Spring/RConn2 -- PS Term Motion v/LConn1
  PS-Simulink Converter1/LConn1 -- Force Spring/RConn2
  Force Spring/LConn1 -- C/RConn1
  Displacement Spring/RConn1 -- Force Spring/RConn1 -- Spring/RConn1
  Displacement Spring/LConn1 -- Spring/LConn1 -- R/RConn1

== system sm_car/Vehicle/Vehicle/Chassis/Spring/Independent/Spring L1/Linear ==
  note: Sensing
  Ctrl : Inport
  Displacement Spring : fl_lib/Mechanical/Mechanical Sensors/Ideal Translational Motion Sensor  reference=foundation.enum.MeasurementReference.difference  acceleration_port=false  velocity_port=true  position_port=true  offset=spr_len0 m
  Force Spring : fl_lib/Mechanical/Mechanical Sensors/Ideal Force Sensor
  PS Term Motion v : fl_lib/Physical Signals/Sinks/PS Terminator
  PS-Simulink Converter : nesl_utility/PS-Simulink Converter  PhysicalDomain=network_engine_domain  SubClassName=ps_output  LeftPortType=input  RightPortType=output  PseudoPeriodic=off  Frequencies=[]  VectorFormat=1-D array  Unit=m  AffineConversion=off
  PS-Simulink Converter1 : nesl_utility/PS-Simulink Converter  PhysicalDomain=network_engine_domain  SubClassName=ps_output  LeftPortType=input  RightPortType=output  PseudoPeriodic=off  Frequencies=[]  VectorFormat=1-D array  Unit=N  AffineConversion=off
  Spring : fl_lib/Mechanical/Translational Elements/Translational Spring  spr_rate=spr_k N/m  v_specify=off  v_priority=None  v=0 m/s  v_nominal_specify=off  v_nominal_value=1  v_nominal_unit=m/s  f_specify=off  f_priority=High  f=-spr_frc0 N  f_nominal_specify=off  f_nominal_value=1  f_nominal_unit=N  x_specify=on  x_priority=High  x=-spr_def0 m  x_nominal_specify=off  x_nominal_value=1  x_nominal_unit=m
  Terminator : Terminator
  R : PMIOPort  Side=Left
  C : PMIOPort  Port=2  Side=Right
  Out Bus Element : Outport  VectorParamsAs1DForOutWhenUnconnected=off  PortName=meas  Element=xSpring
  Out Bus Element1 : Outport  VectorParamsAs1DForOutWhenUnconnected=off  PortName=meas  Element=FSpring
  wires:
  PS-Simulink Converter1/1 -> Out Bus Element1/1
  Ctrl/1 -> Terminator/1
  PS-Simulink Converter/1 -> Out Bus Element/1
  connections:
  Spring/LConn1 -- R/RConn1 -- Displacement Spring/LConn1
  Spring/RConn1 -- Force Spring/RConn1 -- Displacement Spring/RConn1
  Force Spring/LConn1 -- C/RConn1
  PS-Simulink Converter1/LConn1 -- Force Spring/RConn2
  Displacement Spring/RConn2 -- PS Term Motion v/LConn1
  Displacement Spring/RConn3 -- PS-Simulink Converter/LConn1

== system sm_car/Vehicle/Vehicle/Chassis/Spring/Independent/Spring L2/Linear ==
  note: Sensing
  Ctrl : Inport
  Displacement Spring : fl_lib/Mechanical/Mechanical Sensors/Ideal Translational Motion Sensor  reference=foundation.enum.MeasurementReference.difference  acceleration_port=false  velocity_port=true  position_port=true  offset=spr_len0 m
  Force Spring : fl_lib/Mechanical/Mechanical Sensors/Ideal Force Sensor
  PS Term Motion v : fl_lib/Physical Signals/Sinks/PS Terminator
  PS-Simulink Converter : nesl_utility/PS-Simulink Converter  PhysicalDomain=network_engine_domain  SubClassName=ps_output  LeftPortType=input  RightPortType=output  PseudoPeriodic=off  Frequencies=[]  VectorFormat=1-D array  Unit=m  AffineConversion=off
  PS-Simulink Converter1 : nesl_utility/PS-Simulink Converter  PhysicalDomain=network_engine_domain  SubClassName=ps_output  LeftPortType=input  RightPortType=output  PseudoPeriodic=off  Frequencies=[]  VectorFormat=1-D array  Unit=N  AffineConversion=off
  Spring : fl_lib/Mechanical/Translational Elements/Translational Spring  spr_rate=spr_k N/m  v_specify=off  v_priority=None  v=0 m/s  v_nominal_specify=off  v_nominal_value=1  v_nominal_unit=m/s  f_specify=off  f_priority=High  f=-spr_frc0 N  f_nominal_specify=off  f_nominal_value=1  f_nominal_unit=N  x_specify=on  x_priority=High  x=-spr_def0 m  x_nominal_specify=off  x_nominal_value=1  x_nominal_unit=m
  Terminator : Terminator
  R : PMIOPort  Side=Left
  C : PMIOPort  Port=2  Side=Right
  Out Bus Element : Outport  VectorParamsAs1DForOutWhenUnconnected=off  PortName=meas  Element=xSpring
  Out Bus Element1 : Outport  VectorParamsAs1DForOutWhenUnconnected=off  PortName=meas  Element=FSpring
  wires:
  PS-Simulink Converter1/1 -> Out Bus Element1/1
  Ctrl/1 -> Terminator/1
  PS-Simulink Converter/1 -> Out Bus Element/1
  connections:
  Spring/LConn1 -- R/RConn1 -- Displacement Spring/LConn1
  Spring/RConn1 -- Force Spring/RConn1 -- Displacement Spring/RConn1
  Force Spring/LConn1 -- C/RConn1
  PS-Simulink Converter1/LConn1 -- Force Spring/RConn2
  Displacement Spring/RConn2 -- PS Term Motion v/LConn1
  Displacement Spring/RConn3 -- PS-Simulink Converter/LConn1

== system sm_car/Vehicle/Vehicle/Chassis/Spring/Independent/Spring R1/Linear ==
  note: Sensing
  Ctrl : Inport
  Displacement Spring : fl_lib/Mechanical/Mechanical Sensors/Ideal Translational Motion Sensor  reference=foundation.enum.MeasurementReference.difference  acceleration_port=false  velocity_port=true  position_port=true  offset=spr_len0 m
  Force Spring : fl_lib/Mechanical/Mechanical Sensors/Ideal Force Sensor
  PS Term Motion v : fl_lib/Physical Signals/Sinks/PS Terminator
  PS-Simulink Converter : nesl_utility/PS-Simulink Converter  PhysicalDomain=network_engine_domain  SubClassName=ps_output  LeftPortType=input  RightPortType=output  PseudoPeriodic=off  Frequencies=[]  VectorFormat=1-D array  Unit=m  AffineConversion=off
  PS-Simulink Converter1 : nesl_utility/PS-Simulink Converter  PhysicalDomain=network_engine_domain  SubClassName=ps_output  LeftPortType=input  RightPortType=output  PseudoPeriodic=off  Frequencies=[]  VectorFormat=1-D array  Unit=N  AffineConversion=off
  Spring : fl_lib/Mechanical/Translational Elements/Translational Spring  spr_rate=spr_k N/m  v_specify=off  v_priority=None  v=0 m/s  v_nominal_specify=off  v_nominal_value=1  v_nominal_unit=m/s  f_specify=off  f_priority=High  f=-spr_frc0 N  f_nominal_specify=off  f_nominal_value=1  f_nominal_unit=N  x_specify=on  x_priority=High  x=-spr_def0 m  x_nominal_specify=off  x_nominal_value=1  x_nominal_unit=m
  Terminator : Terminator
  R : PMIOPort  Side=Left
  C : PMIOPort  Port=2  Side=Right
  Out Bus Element : Outport  VectorParamsAs1DForOutWhenUnconnected=off  PortName=meas  Element=xSpring
  Out Bus Element1 : Outport  VectorParamsAs1DForOutWhenUnconnected=off  PortName=meas  Element=FSpring
  wires:
  PS-Simulink Converter1/1 -> Out Bus Element1/1
  Ctrl/1 -> Terminator/1
  PS-Simulink Converter/1 -> Out Bus Element/1
  connections:
  Spring/LConn1 -- R/RConn1 -- Displacement Spring/LConn1
  Spring/RConn1 -- Force Spring/RConn1 -- Displacement Spring/RConn1
  Force Spring/LConn1 -- C/RConn1
  PS-Simulink Converter1/LConn1 -- Force Spring/RConn2
  Displacement Spring/RConn2 -- PS Term Motion v/LConn1
  Displacement Spring/RConn3 -- PS-Simulink Converter/LConn1

== system sm_car/Vehicle/Vehicle/Chassis/Spring/Independent/Spring R2/Linear ==
  note: Sensing
  Ctrl : Inport
  Displacement Spring : fl_lib/Mechanical/Mechanical Sensors/Ideal Translational Motion Sensor  reference=foundation.enum.MeasurementReference.difference  acceleration_port=false  velocity_port=true  position_port=true  offset=spr_len0 m
  Force Spring : fl_lib/Mechanical/Mechanical Sensors/Ideal Force Sensor
  PS Term Motion v : fl_lib/Physical Signals/Sinks/PS Terminator
  PS-Simulink Converter : nesl_utility/PS-Simulink Converter  PhysicalDomain=network_engine_domain  SubClassName=ps_output  LeftPortType=input  RightPortType=output  PseudoPeriodic=off  Frequencies=[]  VectorFormat=1-D array  Unit=m  AffineConversion=off
  PS-Simulink Converter1 : nesl_utility/PS-Simulink Converter  PhysicalDomain=network_engine_domain  SubClassName=ps_output  LeftPortType=input  RightPortType=output  PseudoPeriodic=off  Frequencies=[]  VectorFormat=1-D array  Unit=N  AffineConversion=off
  Spring : fl_lib/Mechanical/Translational Elements/Translational Spring  spr_rate=spr_k N/m  v_specify=off  v_priority=None  v=0 m/s  v_nominal_specify=off  v_nominal_value=1  v_nominal_unit=m/s  f_specify=off  f_priority=High  f=-spr_frc0 N  f_nominal_specify=off  f_nominal_value=1  f_nominal_unit=N  x_specify=on  x_priority=High  x=-spr_def0 m  x_nominal_specify=off  x_nominal_value=1  x_nominal_unit=m
  Terminator : Terminator
  R : PMIOPort  Side=Left
  C : PMIOPort  Port=2  Side=Right
  Out Bus Element : Outport  VectorParamsAs1DForOutWhenUnconnected=off  PortName=meas  Element=xSpring
  Out Bus Element1 : Outport  VectorParamsAs1DForOutWhenUnconnected=off  PortName=meas  Element=FSpring
  wires:
  PS-Simulink Converter1/1 -> Out Bus Element1/1
  Ctrl/1 -> Terminator/1
  PS-Simulink Converter/1 -> Out Bus Element/1
  connections:
  Spring/LConn1 -- R/RConn1 -- Displacement Spring/LConn1
  Spring/RConn1 -- Force Spring/RConn1 -- Displacement Spring/RConn1
  Force Spring/LConn1 -- C/RConn1
  PS-Simulink Converter1/LConn1 -- Force Spring/RConn2
  Displacement Spring/RConn2 -- PS Term Motion v/LConn1
  Displacement Spring/RConn3 -- PS-Simulink Converter/LConn1
